simulink model "RRTMS_Arsitektur_Fisik"  (R2026a)
settings: Solver=VariableStepAuto
settings Model: Creator=afifah03  LastModifiedBy=afifah03

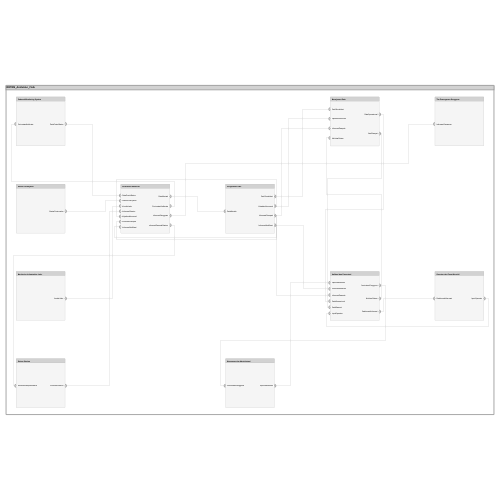
[thumbnail: Simulink's stored preview of the top-level diagram]
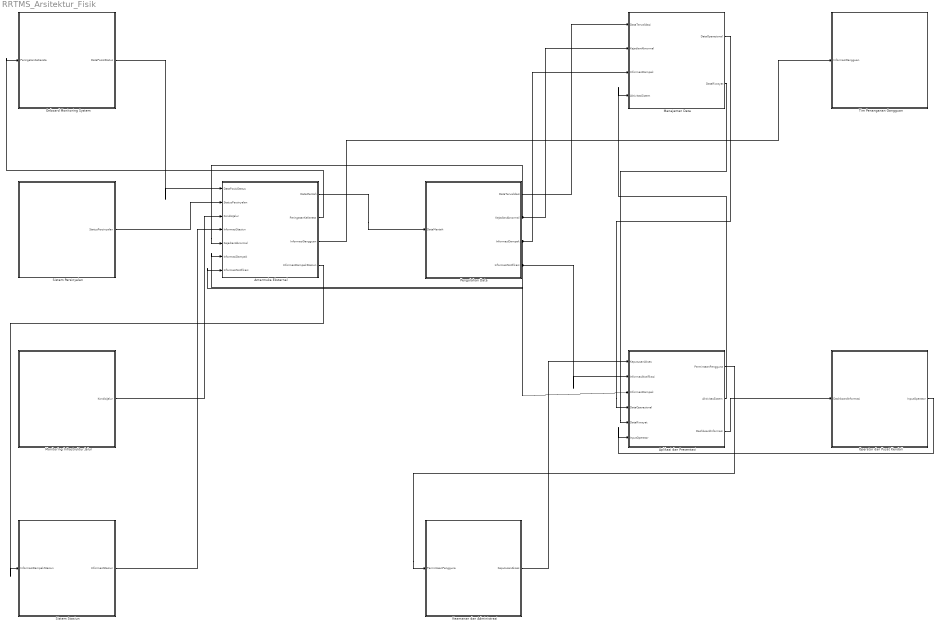
== system RRTMS_Arsitektur_Fisik ==
  Antarmuka Eksternal : Subsystem
      settings: PortSchema="{\"entries\":[{\"content\":{\"headerSize\":26,\"margin\":15,\"minimumSpacing\":25,\"sides\":[{\"content\":{\"connectorIds\":[\"In1\",\"In2\",\"In3\",\"In4\",\"In5\",\"In6\",\"In7\"]},\"type\":\"ConnectorPlacement.EquallySpacedRectSide\",\"uuid\":\"944dc65e-47af-45ed-a139-0647cb5b290a\"},{\"content\":{\"connectorIds\":[\"Out1\",\"Out2\",\"Out3\",\"Out4\"],\"side\":\"RIGHT\"},\"type\":\"ConnectorPlacement.EquallySpacedRectSide\",\"uuid\":\"cbdca632-76b6-4263-a090-790ed7d4bdf6\"},{\"content\":{\"side\":\"TOP\"},\"type\":\"ConnectorPlacement.EquallySpacedRectSide\",\"uuid\":\"9688978b-e9eb-4274-b3ec-2a343f050208\"}]},\"type\":\"ConnectorPlacement.EquallySpacedConnector\",\"uuid\":\"61d49fba-30a1-41fb-88c7-7b17ecf26b87\"}],\"packageUris\":[\"http://schema.mathworks.com/mf0/Connector/R2020b\"],\"version\":\"1.0\"}"
  Aplikasi dan Presentasi : Subsystem
      settings: PortSchema="{\"entries\":[{\"content\":{\"headerSize\":26,\"margin\":15,\"minimumSpacing\":25,\"sides\":[{\"content\":{\"connectorIds\":[\"In1\",\"In2\",\"In3\",\"In4\",\"In5\",\"In6\"]},\"type\":\"ConnectorPlacement.EquallySpacedRectSide\",\"uuid\":\"944dc65e-47af-45ed-a139-0647cb5b290a\"},{\"content\":{\"connectorIds\":[\"Out1\",\"Out2\",\"Out3\"],\"side\":\"RIGHT\"},\"type\":\"ConnectorPlacement.EquallySpacedRectSide\",\"uuid\":\"cbdca632-76b6-4263-a090-790ed7d4bdf6\"},{\"content\":{\"side\":\"TOP\"},\"type\":\"ConnectorPlacement.EquallySpacedRectSide\",\"uuid\":\"9688978b-e9eb-4274-b3ec-2a343f050208\"}]},\"type\":\"ConnectorPlacement.EquallySpacedConnector\",\"uuid\":\"61d49fba-30a1-41fb-88c7-7b17ecf26b87\"}],\"packageUris\":[\"http://schema.mathworks.com/mf0/Connector/R2020b\"],\"version\":\"1.0\"}"
  Keamanan dan Administrasi : Subsystem
      settings: PortSchema="{\"entries\":[{\"content\":{\"headerSize\":26,\"margin\":15,\"minimumSpacing\":25,\"sides\":[{\"content\":{\"connectorIds\":[\"In1\"]},\"type\":\"ConnectorPlacement.EquallySpacedRectSide\",\"uuid\":\"944dc65e-47af-45ed-a139-0647cb5b290a\"},{\"content\":{\"connectorIds\":[\"Out1\"],\"side\":\"RIGHT\"},\"type\":\"ConnectorPlacement.EquallySpacedRectSide\",\"uuid\":\"cbdca632-76b6-4263-a090-790ed7d4bdf6\"},{\"content\":{\"side\":\"TOP\"},\"type\":\"ConnectorPlacement.EquallySpacedRectSide\",\"uuid\":\"9688978b-e9eb-4274-b3ec-2a343f050208\"}]},\"type\":\"ConnectorPlacement.EquallySpacedConnector\",\"uuid\":\"61d49fba-30a1-41fb-88c7-7b17ecf26b87\"}],\"packageUris\":[\"http://schema.mathworks.com/mf0/Connector/R2020b\"],\"version\":\"1.0\"}"
  Manajemen Data : Subsystem
      settings: PortSchema="{\"entries\":[{\"content\":{\"headerSize\":26,\"margin\":15,\"minimumSpacing\":25,\"sides\":[{\"content\":{\"connectorIds\":[\"In1\",\"In2\",\"In3\",\"In4\"]},\"type\":\"ConnectorPlacement.EquallySpacedRectSide\",\"uuid\":\"944dc65e-47af-45ed-a139-0647cb5b290a\"},{\"content\":{\"connectorIds\":[\"Out1\",\"Out2\"],\"side\":\"RIGHT\"},\"type\":\"ConnectorPlacement.EquallySpacedRectSide\",\"uuid\":\"cbdca632-76b6-4263-a090-790ed7d4bdf6\"},{\"content\":{\"side\":\"TOP\"},\"type\":\"ConnectorPlacement.EquallySpacedRectSide\",\"uuid\":\"9688978b-e9eb-4274-b3ec-2a343f050208\"}]},\"type\":\"ConnectorPlacement.EquallySpacedConnector\",\"uuid\":\"61d49fba-30a1-41fb-88c7-7b17ecf26b87\"}],\"packageUris\":[\"http://schema.mathworks.com/mf0/Connector/R2020b\"],\"version\":\"1.0\"}"
  Monitoring Infrastruktur Jalur : Subsystem
      settings: PortSchema="{\"entries\":[{\"content\":{\"headerSize\":26,\"margin\":15,\"minimumSpacing\":25,\"sides\":[{\"content\":{},\"type\":\"ConnectorPlacement.EquallySpacedRectSide\",\"uuid\":\"944dc65e-47af-45ed-a139-0647cb5b290a\"},{\"content\":{\"connectorIds\":[\"Out1\"],\"side\":\"RIGHT\"},\"type\":\"ConnectorPlacement.EquallySpacedRectSide\",\"uuid\":\"cbdca632-76b6-4263-a090-790ed7d4bdf6\"},{\"content\":{\"side\":\"TOP\"},\"type\":\"ConnectorPlacement.EquallySpacedRectSide\",\"uuid\":\"9688978b-e9eb-4274-b3ec-2a343f050208\"}]},\"type\":\"ConnectorPlacement.EquallySpacedConnector\",\"uuid\":\"61d49fba-30a1-41fb-88c7-7b17ecf26b87\"}],\"packageUris\":[\"http://schema.mathworks.com/mf0/Connector/R2020b\"],\"version\":\"1.0\"}"
  Onboard Monitoring System : Subsystem
      settings: PortSchema="{\"entries\":[{\"content\":{\"headerSize\":26,\"margin\":15,\"minimumSpacing\":25,\"sides\":[{\"content\":{\"connectorIds\":[\"In1\"]},\"type\":\"ConnectorPlacement.EquallySpacedRectSide\",\"uuid\":\"944dc65e-47af-45ed-a139-0647cb5b290a\"},{\"content\":{\"connectorIds\":[\"Out1\"],\"side\":\"RIGHT\"},\"type\":\"ConnectorPlacement.EquallySpacedRectSide\",\"uuid\":\"cbdca632-76b6-4263-a090-790ed7d4bdf6\"},{\"content\":{\"side\":\"TOP\"},\"type\":\"ConnectorPlacement.EquallySpacedRectSide\",\"uuid\":\"9688978b-e9eb-4274-b3ec-2a343f050208\"}]},\"type\":\"ConnectorPlacement.EquallySpacedConnector\",\"uuid\":\"61d49fba-30a1-41fb-88c7-7b17ecf26b87\"}],\"packageUris\":[\"http://schema.mathworks.com/mf0/Connector/R2020b\"],\"version\":\"1.0\"}"
  Operator dan Pusat Kendali : Subsystem
      settings: PortSchema="{\"entries\":[{\"content\":{\"headerSize\":26,\"margin\":15,\"minimumSpacing\":25,\"sides\":[{\"content\":{\"connectorIds\":[\"In1\"]},\"type\":\"ConnectorPlacement.EquallySpacedRectSide\",\"uuid\":\"944dc65e-47af-45ed-a139-0647cb5b290a\"},{\"content\":{\"connectorIds\":[\"Out1\"],\"side\":\"RIGHT\"},\"type\":\"ConnectorPlacement.EquallySpacedRectSide\",\"uuid\":\"cbdca632-76b6-4263-a090-790ed7d4bdf6\"},{\"content\":{\"side\":\"TOP\"},\"type\":\"ConnectorPlacement.EquallySpacedRectSide\",\"uuid\":\"9688978b-e9eb-4274-b3ec-2a343f050208\"}]},\"type\":\"ConnectorPlacement.EquallySpacedConnector\",\"uuid\":\"61d49fba-30a1-41fb-88c7-7b17ecf26b87\"}],\"packageUris\":[\"http://schema.mathworks.com/mf0/Connector/R2020b\"],\"version\":\"1.0\"}"
  Pengolahan Data : Subsystem
      settings: PortSchema="{\"entries\":[{\"content\":{\"headerSize\":26,\"margin\":15,\"minimumSpacing\":25,\"sides\":[{\"content\":{\"connectorIds\":[\"In1\"]},\"type\":\"ConnectorPlacement.EquallySpacedRectSide\",\"uuid\":\"944dc65e-47af-45ed-a139-0647cb5b290a\"},{\"content\":{\"connectorIds\":[\"Out1\",\"Out2\",\"Out3\",\"Out4\"],\"side\":\"RIGHT\"},\"type\":\"ConnectorPlacement.EquallySpacedRectSide\",\"uuid\":\"cbdca632-76b6-4263-a090-790ed7d4bdf6\"},{\"content\":{\"side\":\"TOP\"},\"type\":\"ConnectorPlacement.EquallySpacedRectSide\",\"uuid\":\"9688978b-e9eb-4274-b3ec-2a343f050208\"}]},\"type\":\"ConnectorPlacement.EquallySpacedConnector\",\"uuid\":\"61d49fba-30a1-41fb-88c7-7b17ecf26b87\"}],\"packageUris\":[\"http://schema.mathworks.com/mf0/Connector/R2020b\"],\"version\":\"1.0\"}"
  Sistem Persinyalan : Subsystem
      settings: PortSchema="{\"entries\":[{\"content\":{\"headerSize\":26,\"margin\":15,\"minimumSpacing\":25,\"sides\":[{\"content\":{},\"type\":\"ConnectorPlacement.EquallySpacedRectSide\",\"uuid\":\"944dc65e-47af-45ed-a139-0647cb5b290a\"},{\"content\":{\"connectorIds\":[\"Out1\"],\"side\":\"RIGHT\"},\"type\":\"ConnectorPlacement.EquallySpacedRectSide\",\"uuid\":\"cbdca632-76b6-4263-a090-790ed7d4bdf6\"},{\"content\":{\"side\":\"TOP\"},\"type\":\"ConnectorPlacement.EquallySpacedRectSide\",\"uuid\":\"9688978b-e9eb-4274-b3ec-2a343f050208\"}]},\"type\":\"ConnectorPlacement.EquallySpacedConnector\",\"uuid\":\"61d49fba-30a1-41fb-88c7-7b17ecf26b87\"}],\"packageUris\":[\"http://schema.mathworks.com/mf0/Connector/R2020b\"],\"version\":\"1.0\"}"
  Sistem Stasiun : Subsystem
      settings: PortSchema="{\"entries\":[{\"content\":{\"headerSize\":26,\"margin\":15,\"minimumSpacing\":25,\"sides\":[{\"content\":{\"connectorIds\":[\"In1\"]},\"type\":\"ConnectorPlacement.EquallySpacedRectSide\",\"uuid\":\"944dc65e-47af-45ed-a139-0647cb5b290a\"},{\"content\":{\"connectorIds\":[\"Out1\"],\"side\":\"RIGHT\"},\"type\":\"ConnectorPlacement.EquallySpacedRectSide\",\"uuid\":\"cbdca632-76b6-4263-a090-790ed7d4bdf6\"},{\"content\":{\"side\":\"TOP\"},\"type\":\"ConnectorPlacement.EquallySpacedRectSide\",\"uuid\":\"9688978b-e9eb-4274-b3ec-2a343f050208\"}]},\"type\":\"ConnectorPlacement.EquallySpacedConnector\",\"uuid\":\"61d49fba-30a1-41fb-88c7-7b17ecf26b87\"}],\"packageUris\":[\"http://schema.mathworks.com/mf0/Connector/R2020b\"],\"version\":\"1.0\"}"
  Tim Penanganan Gangguan : Subsystem
      settings: PortSchema="{\"entries\":[{\"content\":{\"headerSize\":26,\"margin\":15,\"minimumSpacing\":25,\"sides\":[{\"content\":{\"connectorIds\":[\"In1\"]},\"type\":\"ConnectorPlacement.EquallySpacedRectSide\",\"uuid\":\"944dc65e-47af-45ed-a139-0647cb5b290a\"},{\"content\":{\"side\":\"RIGHT\"},\"type\":\"ConnectorPlacement.EquallySpacedRectSide\",\"uuid\":\"cbdca632-76b6-4263-a090-790ed7d4bdf6\"},{\"content\":{\"side\":\"TOP\"},\"type\":\"ConnectorPlacement.EquallySpacedRectSide\",\"uuid\":\"9688978b-e9eb-4274-b3ec-2a343f050208\"}]},\"type\":\"ConnectorPlacement.EquallySpacedConnector\",\"uuid\":\"61d49fba-30a1-41fb-88c7-7b17ecf26b87\"}],\"packageUris\":[\"http://schema.mathworks.com/mf0/Connector/R2020b\"],\"version\":\"1.0\"}"
  wires:
  Onboard Monitoring System/1(DataPosisiStatus) -> Antarmuka Eksternal/1(DataPosisiStatus)
  Sistem Persinyalan/1(StatusPersinyalan) -> Antarmuka Eksternal/2(StatusPersinyalan)
  Monitoring Infrastruktur Jalur/1(KondisiJalur) -> Antarmuka Eksternal/3(KondisiJalur)
  Sistem Stasiun/1(InformasiStasiun) -> Antarmuka Eksternal/4(InformasiStasiun)
  Antarmuka Eksternal/1(DataMentah) -> Pengolahan Data/1(DataMentah)
  Pengolahan Data/1(DataTervalidasi) -> Manajemen Data/1(DataTervalidasi)
  Pengolahan Data/2(KejadianAbnormal) -> Manajemen Data/2(KejadianAbnormal), Antarmuka Eksternal/5(KejadianAbnormal)
  Pengolahan Data/3(InformasiDampak) -> Manajemen Data/3(InformasiDampak), Aplikasi dan Presentasi/3(InformasiDampak), Antarmuka Eksternal/6(InformasiDampak)
  Pengolahan Data/4(InformasiNotifikasi) -> Aplikasi dan Presentasi/2(InformasiNotifikasi), Antarmuka Eksternal/7(InformasiNotifikasi)
  Manajemen Data/1(DataOperasional) -> Aplikasi dan Presentasi/4(DataOperasional)
  Manajemen Data/2(DataRiwayat) -> Aplikasi dan Presentasi/5(DataRiwayat)
  Aplikasi dan Presentasi/2(AktivitasSistem) -> Manajemen Data/4(AktivitasSistem)
  Aplikasi dan Presentasi/1(PermintaanPengguna) -> Keamanan dan Administrasi/1(PermintaanPengguna)
  Keamanan dan Administrasi/1(KeputusanAkses) -> Aplikasi dan Presentasi/1(KeputusanAkses)
  Antarmuka Eksternal/2(PeringatanKeKereta) -> Onboard Monitoring System/1(PeringatanKeKereta)
  Antarmuka Eksternal/3(InformasiGangguan) -> Tim Penanganan Gangguan/1(InformasiGangguan)
  Antarmuka Eksternal/4(InformasiDampakStasiun) -> Sistem Stasiun/1(InformasiDampakStasiun)
  Aplikasi dan Presentasi/3(DashboardInformasi) -> Operator dan Pusat Kendali/1(DashboardInformasi)
  Operator dan Pusat Kendali/1(InputOperator) -> Aplikasi dan Presentasi/6(InputOperator)

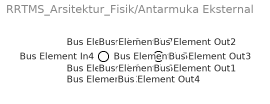
== system RRTMS_Arsitektur_Fisik/Antarmuka Eksternal ==
  Bus Element In1 : Inport  PortName=DataPosisiStatus
  Bus Element In2 : Inport  Port=2  PortName=StatusPersinyalan
  Bus Element In3 : Inport  Port=3  PortName=KondisiJalur
  Bus Element In4 : Inport  Port=4  PortName=InformasiStasiun
  Bus Element In5 : Inport  Port=5  PortName=KejadianAbnormal
  Bus Element In6 : Inport  Port=6  PortName=InformasiDampak
  Bus Element In7 : Inport  Port=7  PortName=InformasiNotifikasi
  Bus Element Out1 : Outport  PortName=DataMentah
  Bus Element Out2 : Outport  Port=2  PortName=PeringatanKeKereta
  Bus Element Out3 : Outport  Port=3  PortName=InformasiGangguan
  Bus Element Out4 : Outport  Port=4  PortName=InformasiDampakStasiun

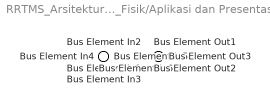
== system RRTMS_Arsitektur_Fisik/Aplikasi dan Presentasi ==
  Bus Element In1 : Inport  PortName=KeputusanAkses
  Bus Element In2 : Inport  Port=2  PortName=InformasiNotifikasi
  Bus Element In3 : Inport  Port=3  PortName=InformasiDampak
  Bus Element In4 : Inport  Port=4  PortName=DataOperasional
  Bus Element In5 : Inport  Port=5  PortName=DataRiwayat
  Bus Element In6 : Inport  Port=6  PortName=InputOperator
  Bus Element Out1 : Outport  PortName=PermintaanPengguna
  Bus Element Out2 : Outport  Port=2  PortName=AktivitasSistem
  Bus Element Out3 : Outport  Port=3  PortName=DashboardInformasi

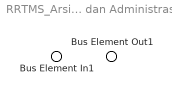
== system RRTMS_Arsitektur_Fisik/Keamanan dan Administrasi ==
  Bus Element In1 : Inport  PortName=PermintaanPengguna
  Bus Element Out1 : Outport  PortName=KeputusanAkses

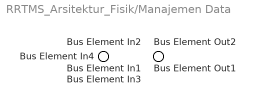
== system RRTMS_Arsitektur_Fisik/Manajemen Data ==
  Bus Element In1 : Inport  PortName=DataTervalidasi
  Bus Element In2 : Inport  Port=2  PortName=KejadianAbnormal
  Bus Element In3 : Inport  Port=3  PortName=InformasiDampak
  Bus Element In4 : Inport  Port=4  PortName=AktivitasSistem
  Bus Element Out1 : Outport  PortName=DataOperasional
  Bus Element Out2 : Outport  Port=2  PortName=DataRiwayat

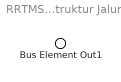
== system RRTMS_Arsitektur_Fisik/Monitoring Infrastruktur Jalur ==
  Bus Element Out1 : Outport  PortName=KondisiJalur

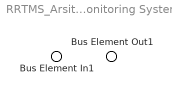
== system RRTMS_Arsitektur_Fisik/Onboard Monitoring System ==
  Bus Element In1 : Inport  PortName=PeringatanKeKereta
  Bus Element Out1 : Outport  PortName=DataPosisiStatus

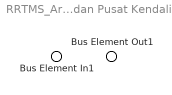
== system RRTMS_Arsitektur_Fisik/Operator dan Pusat Kendali ==
  Bus Element In1 : Inport  PortName=DashboardInformasi
  Bus Element Out1 : Outport  PortName=InputOperator

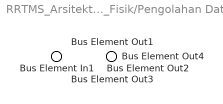
== system RRTMS_Arsitektur_Fisik/Pengolahan Data ==
  Bus Element In1 : Inport  PortName=DataMentah
  Bus Element Out1 : Outport  PortName=DataTervalidasi
  Bus Element Out2 : Outport  Port=2  PortName=KejadianAbnormal
  Bus Element Out3 : Outport  Port=3  PortName=InformasiDampak
  Bus Element Out4 : Outport  Port=4  PortName=InformasiNotifikasi

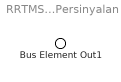
== system RRTMS_Arsitektur_Fisik/Sistem Persinyalan ==
  Bus Element Out1 : Outport  PortName=StatusPersinyalan

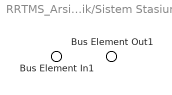
== system RRTMS_Arsitektur_Fisik/Sistem Stasiun ==
  Bus Element In1 : Inport  PortName=InformasiDampakStasiun
  Bus Element Out1 : Outport  PortName=InformasiStasiun

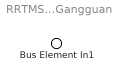
== system RRTMS_Arsitektur_Fisik/Tim Penanganan Gangguan ==
  Bus Element In1 : Inport  PortName=InformasiGangguan
